simulink model "tb_perception"  (R2026b)
undefined symbols (not defined in the file or in its folder): Ts
settings Model: Creator=aomar  LastModifiedBy=aomar

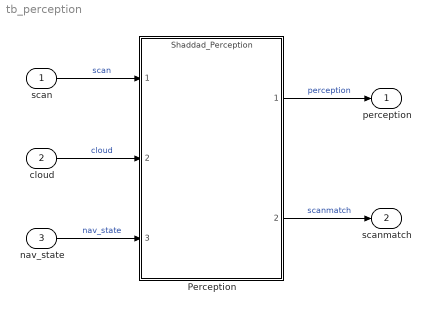
== system tb_perception ==
  scan : Inport  OutDataTypeStr=Bus: Bus_LidarScanRaw  SampleTime=Ts.lidar  Interpolate=off
  cloud : Inport  Port=2  OutDataTypeStr=Bus: Bus_LidarCloudRaw  SampleTime=Ts.lidar  Interpolate=off
  nav_state : Inport  Port=3  OutDataTypeStr=Bus: Bus_NavState  SampleTime=Ts.nav  Interpolate=off
  Perception : ModelReference  ModelNameDialog=Shaddad_Perception  SimulationMode=Normal  ModelReferenceVersion=1.1
  perception : Outport
  scanmatch : Outport  Port=2
  wires:
  scan/1 -> Perception/1  "scan"
  cloud/1 -> Perception/2  "cloud"
  nav_state/1 -> Perception/3  "nav_state"
  Perception/1 -> perception/1  "perception"
  Perception/2 -> scanmatch/1  "scanmatch"
